simulink model "drone"  (R2026b)
settings: Solver=ode4  StopTime=inf  FixedStep=0.01
values from neighbouring files (symbols this model uses):
  A_d = sys_d.A    [controller_observer_design.m]    (also in setup.m)
  B_d = sys_d.B    [controller_observer_design.m]    (also in setup.m)
  C_d = sys_d.C    [controller_observer_design.m]    (also in setup.m)
  K_discrete = dlqr(A_d,B_d,Q*Ts,R*Ts)    [controller_observer_design.m]    (also in setup.m)
  omega2u = [k, k, k, k; L*k, 0, -L*k, 0; 0, L*k, 0, -L*k; b, -b, b, -b]    [controller_observer_design.m]    (also in notes.m; setup.m)
  parameters =     [parameters.mat]
  Ts = 0.01    [controller_observer_design.m]    (also in setup.m)
  u2omega = (1/(4*b*L*k)) * [b*L, 2*b, 0, L*k; b*L, 0, 2*b, -L*k; b*L, -2*b, 0, L*k; b*L, 0, -2*b, -L*k]    [controller_observer_design.m]    (also in notes.m; setup.m)
undefined symbols (not defined in the file or in its folder): L_discrete
libraries: simulink x2
settings Model: Creator=elton  LastModifiedBy=eltnw

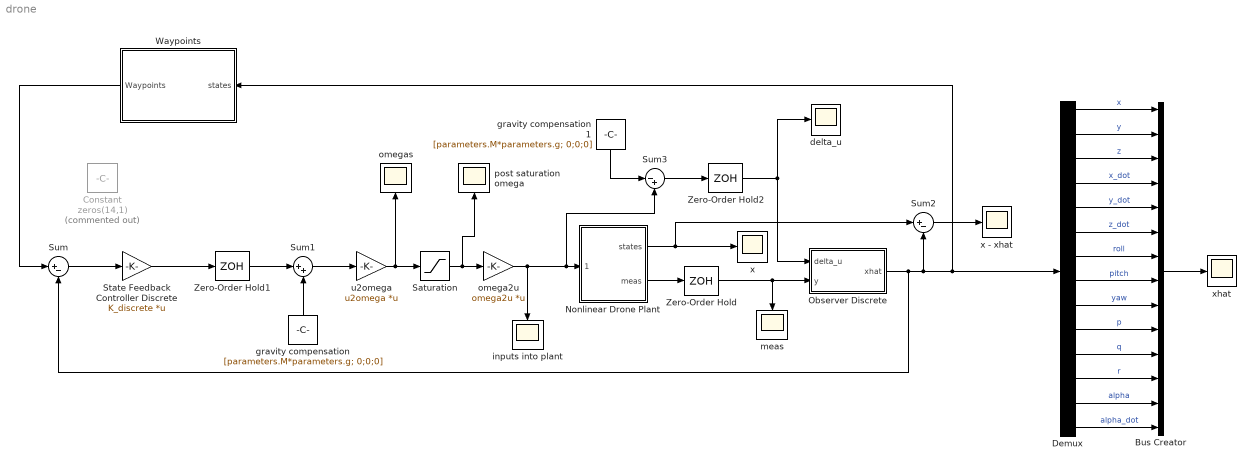
== system drone ==
  Bus Creator : BusCreator  Inputs=14
  Constant : Constant  Commented=on  Value=zeros(14,1)
  Demux : Demux  Outputs=14
  Nonlinear Drone Plant : Subsystem
  Observer Discrete : Subsystem
  Saturation : Saturate  UpperLimit=250000  LowerLimit=-250000
  State Feedback Controller Discrete : Gain  Gain=K_discrete  Multiplication=Matrix(K*u)
  Sum : Sum  Inputs=|+-
  Sum1 : Sum  Inputs=|++
  Sum2 : Sum  Inputs=|+-
  Sum3 : Sum  Inputs=|-+
  Waypoints : Subsystem
  Zero-Order Hold : ZeroOrderHold  SampleTime=Ts
  Zero-Order Hold1 : ZeroOrderHold  SampleTime=Ts
  Zero-Order Hold2 : ZeroOrderHold  SampleTime=Ts
  delta_u : Scope
      settings: ActiveDisplayYMinimum=-0.1401923631580794  ActiveDisplayYMaximum=0.1652403175832419
  gravity compensation : Constant  Value=[parameters.M*parameters.g; 0;0;0]
  gravity compensation1 : Constant  Value=[parameters.M*parameters.g; 0;0;0]
  inputs into plant : Scope
      settings: ActiveDisplayYMinimum=-2.3883084159431922  ActiveDisplayYMaximum=20.39828479264926  DataLoggingVariableName=ScopeData7
  meas : Scope
      settings: ActiveDisplayYMinimum=-955.77756320006051  ActiveDisplayYMaximum=3490.5526217286788
  omega2u : Gain  Gain=omega2u  Multiplication=Matrix(K*u)
  omegas : Scope
      settings: ActiveDisplayYMinimum=-4.7458150182251656E+8  ActiveDisplayYMaximum=6.7744655103517926E+8  DataLoggingVariableName=ScopeData8
  post saturation omega : Scope
      settings: ActiveDisplayYMinimum=-3047.5832245298225  ActiveDisplayYMaximum=278116.39813605888  DataLoggingVariableName=ScopeData9
  u2omega : Gain  Gain=u2omega  Multiplication=Matrix(K*u)
  x : Scope
      settings: ActiveDisplayYMinimum=-2.3057854953189612  ActiveDisplayYMaximum=11.36705971645924  DataLoggingVariableName=ScopeData6
  x - xhat : Scope
      settings: ActiveDisplayYMinimum=-0.016053555537243414  ActiveDisplayYMaximum=0.016145822671605803  DataLoggingVariableName=ScopeData2
  xhat : Scope
      settings: ActiveDisplayYMinimum=-1.314265661412086  ActiveDisplayYMaximum=11.256891286390609  DataLoggingVariableName=ScopeData3
  wires:
  Sum/1 -> State Feedback Controller Discrete/1
  omega2u/1 -> Sum3/2, Nonlinear Drone Plant/1(inputs), inputs into plant/1
  Nonlinear Drone Plant/1(states) -> x/1, Sum2/1
  Zero-Order Hold1/1 -> Sum1/1
  Nonlinear Drone Plant/2(meas) -> Zero-Order Hold/1
  u2omega/1 -> Saturation/1, omegas/1
  Saturation/1 -> post saturation omega/1, omega2u/1
  Zero-Order Hold/1 -> meas/1, Observer Discrete/2(y)
  Zero-Order Hold2/1 -> delta_u/1, Observer Discrete/1(delta_u)
  Observer Discrete/1(xhat) -> Waypoints/1(states), Demux/1, Sum2/2, Sum/2
  Sum2/1 -> x - xhat/1
  gravity compensation/1 -> Sum1/2
  State Feedback Controller Discrete/1 -> Zero-Order Hold1/1
  gravity compensation1/1 -> Sum3/1
  Sum1/1 -> u2omega/1
  Sum3/1 -> Zero-Order Hold2/1
  Waypoints/1(Waypoints) -> Sum/1
  Demux/1 -> Bus Creator/1  "x"
  Demux/2 -> Bus Creator/2  "y"
  Demux/3 -> Bus Creator/3  "z"
  Demux/4 -> Bus Creator/4  "x_dot"
  Demux/5 -> Bus Creator/5  "y_dot"
  Demux/6 -> Bus Creator/6  "z_dot"
  Demux/7 -> Bus Creator/7  "roll"
  Demux/8 -> Bus Creator/8  "pitch"
  Demux/9 -> Bus Creator/9  "yaw"
  Demux/10 -> Bus Creator/10  "p"
  Demux/11 -> Bus Creator/11  "q"
  Demux/12 -> Bus Creator/12  "r"
  Demux/13 -> Bus Creator/13  "alpha"
  Demux/14 -> Bus Creator/14  "alpha_dot"
  Bus Creator/1 -> xhat/1

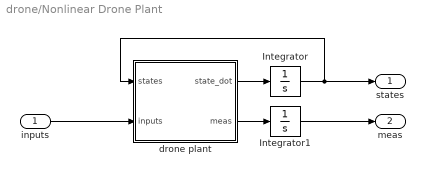
== system drone/Nonlinear Drone Plant ==
  inputs : Inport
  Integrator : Integrator  InitialCondition=[zeros(12,1); 0; 0]
  Integrator1 : Integrator  InitialCondition=zeros(6,1)
  drone plant : MATLAB Function  TreatAsAtomicUnit=on
  states : Outport
  meas : Outport  Port=2
  wires:
  drone plant/1(state_dot) -> Integrator/1
  Integrator/1 -> states/1, drone plant/1(states)
  inputs/1 -> drone plant/2(inputs)
  Integrator1/1 -> meas/1
  drone plant/2(meas) -> Integrator1/1

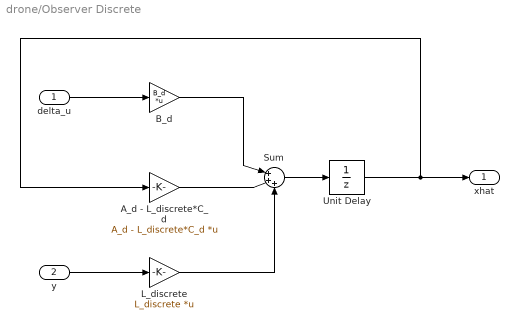
== system drone/Observer Discrete ==
  delta_u : Inport
  y : Inport  Port=2
  A_d - L_discrete*C_d : Gain  Gain=A_d - L_discrete*C_d  Multiplication=Matrix(K*u)
  B_d : Gain  Gain=B_d  Multiplication=Matrix(K*u)
  L_discrete : Gain  Gain=L_discrete  Multiplication=Matrix(K*u)
  Sum : Sum  Inputs=|+++
  Unit Delay : UnitDelay  InitialCondition=zeros(14,1)  SampleTime=-1
  xhat : Outport
  wires:
  y/1 -> L_discrete/1
  B_d/1 -> Sum/1
  L_discrete/1 -> Sum/3
  A_d - L_discrete*C_d/1 -> Sum/2
  Sum/1 -> Unit Delay/1
  Unit Delay/1 -> A_d - L_discrete*C_d/1, xhat/1
  delta_u/1 -> B_d/1

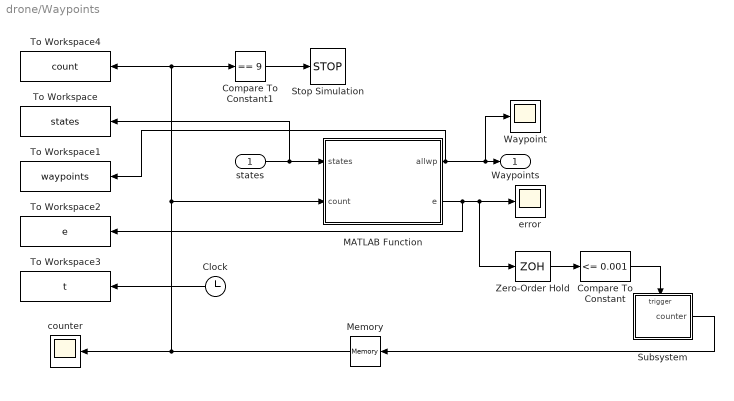
== system drone/Waypoints ==
  states : Inport
  Clock : Clock
  Compare To Constant : simulink/Logic and Bit Operations/Compare To Constant  relop=<=  const=0.001  OutDataTypeStr=boolean
  Compare To Constant1 : simulink/Logic and Bit Operations/Compare To Constant  relop===  const=9  OutDataTypeStr=boolean
  MATLAB Function : MATLAB Function  TreatAsAtomicUnit=on
  Memory : Memory  InheritSampleTime=on
  Stop Simulation : Stop
  Subsystem : Subsystem
  To Workspace : ToWorkspace  VariableName=states  SampleTime=-1
  To Workspace1 : ToWorkspace  VariableName=waypoints  SampleTime=-1
  To Workspace2 : ToWorkspace  VariableName=e  SampleTime=-1
  To Workspace3 : ToWorkspace  VariableName=t  SampleTime=-1
  To Workspace4 : ToWorkspace  VariableName=count  SampleTime=-1
  Waypoint : Scope
      settings: DataLoggingVariableName=ScopeData4
  Zero-Order Hold : ZeroOrderHold  SampleTime=0.01
  counter : Scope
      settings: DataLoggingVariableName=ScopeData5
  error : Scope
      settings: ActiveDisplayYMinimum=-0.89185486903848621  ActiveDisplayYMaximum=8.0341746816232842  DataLoggingVariableName=ScopeData10
  Waypoints : Outport
  wires:
  Compare To Constant/1 -> Subsystem/Trigger
  Memory/1 -> Compare To Constant1/1, To Workspace4/1, MATLAB Function/2(count), counter/1
  MATLAB Function/2(e) -> To Workspace2/1, Zero-Order Hold/1, error/1
  states/1 -> To Workspace/1, MATLAB Function/1(states)
  Subsystem/1(counter) -> Memory/1
  Zero-Order Hold/1 -> Compare To Constant/1
  Clock/1 -> To Workspace3/1
  MATLAB Function/1(allwp) -> To Workspace1/1, Waypoint/1, Waypoints/1
  Compare To Constant1/1 -> Stop Simulation/1

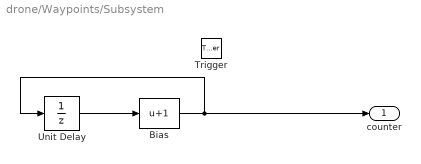
== system drone/Waypoints/Subsystem ==
  Trigger : TriggerPort  VariantControl=(inherit)  InitialTriggerSignalState=positive  PortDimensions=1
  Bias : Bias  Bias=1  SaturateOnIntegerOverflow=off
  Unit Delay : UnitDelay  SampleTime=-1
  counter : Outport
  wires:
  Unit Delay/1 -> Bias/1
  Bias/1 -> Unit Delay/1, counter/1

== matlab function drone/Waypoints/MATLAB Function ==
  data: states input; allwp output; count input; e output
function [allwp, e] = waypoints(states, count)
wps0 = [5 8 8 7 9 6 3 3;
    1 3 2 9 6 5 8 2;
    1 5 9 10 5 4 3 3];

%wps0 = [4 10 0 1 7 2 8 10;
        %2 9 8 5 2 1 8 9;
        %8 4 9 7 5 3 1 1];
persistent wps
if isempty(wps)
    wps = shortestTour(wps0, zeros(3,1), zeros(3,1));
end
%wps = wps0;
xi = states(1:3);
wp = zeros(3,1);
if count < size(wps, 2)
    wp = wps(:, uint8(count+1));
end
e = norm(xi - wp);
d_max = 0.7;
err  = wp - xi;
dist = norm(err);
if dist > d_max
    ref = xi + d_max * err / dist;
else
    ref = wp;
end
allwp = zeros(14,1);
allwp(1:3) = ref;
end

function out = shortestTour(P, startPt, endPt)
N  = size(P, 2);
nm = 2^N;

D = zeros(N, N);
for i = 1:N
    for j = 1:N
        D(i,j) = norm(P(:,i) - P(:,j));
    end
end

% Length of the order as entered
givenLen = norm(P(:,1) - startPt) + norm(P(:,N) - endPt);
for i = 1:N-1
    givenLen = givenLen + D(i,i+1);
end

% Held-Karp: exact shortest path start -> all points -> end
cost   = inf(nm, N);
parent = zeros(nm, N);
for j = 1:N
    cost(2^(j-1) + 1, j) = norm(P(:,j) - startPt);
end
for mask = 1:nm-1
    for j = 1:N
        if bitand(mask, 2^(j-1)) == 0 || isinf(cost(mask+1, j))
            continue;
        end
        for k = 1:N
            if bitand(mask, 2^(k-1)) ~= 0
                continue;
            end
            nmask = mask + 2^(k-1);
            c = cost(mask+1, j) + D(j,k);
            if c < cost(nmask+1, k)
                cost(nmask+1, k)   = c;
                parent(nmask+1, k) = j;
            end
        end
    end
end

allMask = nm - 1;
best = inf;
last = 1;
for j = 1:N
    c = cost(allMask+1, j) + norm(P(:,j) - endPt);
    if c < best
        best = c;
        last = j;
    end
end

% Already shortest (including ties)? Keep the entered order.
if givenLen <= best + 1e-9
    out = P;
    return;
end

order = zeros(1, N);
mask  = allMask;
j     = last;
for idx = N:-1:1
    order(idx) = j;
    pj   = parent(mask+1, j);
    mask = mask - 2^(j-1);
    j    = pj;
end
out = P(:, order);
end

== matlab function drone/Nonlinear Drone Plant/drone plant ==
  data: states input size=14; inputs input size=4; state_dot output size=14; parameters parameter; meas output
%% non-linear state space
function [state_dot, meas]  = nonlin_state_space(states, inputs, parameters)
m     = parameters.m;
m_p    = parameters.m_p;
M     = m + m_p;
g     = parameters.g;
l     = parameters.l;
k_D    = parameters.k_D;
I_xx  = parameters.I_xx;
I_yy  = parameters.I_yy;
I_zz  = parameters.I_zz;

xi = states(1:3);
xi_dot = states(4:6);
eta = states(7:9);
nu = states(10:12);
alpha = states(13);
alpha_dot = states(14);

u_T = inputs(1);
tau = inputs(2:4);

x_dot = xi_dot(1);
y_dot = xi_dot(2);
z_dot = xi_dot(3);

% kinematics
phi = eta(1);
theta = eta(2);
psi = eta(3);
W_inv = [1,  sin(phi)*tan(theta), cos(phi)*tan(theta);
    0,  cos(phi),            -sin(phi);
    0,  sin(phi)/cos(theta), cos(phi)/cos(theta)];

eta_dot = W_inv*nu;

%rotational dynamics
p_dot = (tau(1)/I_xx) + ((I_yy-I_zz)/I_xx)*nu(2)*nu(3);
q_dot = (tau(2)/I_yy) + ((I_zz-I_xx)/I_yy)*nu(1)*nu(3);
r_dot = (tau(3)/I_zz) + ((I_xx-I_yy)/I_zz)*nu(1)*nu(2);
nu_dot = [p_dot; q_dot; r_dot];

%translational dynamics
c_alpha = cos(alpha);
s_alpha = sin(alpha);
c_phi = cos(phi); s_phi = sin(phi);
c_theta = cos(theta); s_theta = sin(theta);
c_psi = cos(psi); s_psi = sin(psi);

Fx = (c_psi*s_theta*c_phi + s_psi*s_phi) * u_T;
Fy = (s_psi*s_theta*c_phi - c_psi*s_phi) * u_T;
Fz = c_theta*c_phi * u_T;

x_dotdot = (1/(m*M)) * ( (m + m_p*c_alpha^2)*(Fx - k_D*x_dot) - m_p*s_alpha*c_alpha*(Fz - k_D*z_dot) + m*m_p*l*alpha_dot^2*s_alpha );
y_dotdot = (Fy - k_D*y_dot) / m;
z_dotdot = (1/(m*M)) * ( (m + m_p*s_alpha^2)*(Fz - k_D*z_dot) - m_p*s_alpha*c_alpha*(Fx - k_D*x_dot) + m*m_p*l*alpha_dot^2*c_alpha ) - g;
xi_dotdot = [x_dotdot; y_dotdot; z_dotdot];

% pendulum dynamics
%alpha_dotdot = (1 / (M * l)) * ( -Fx * c_alpha + Fz * s_alpha + k_D * x_dot * c_alpha - k_D * z_dot * s_alpha );
alpha_dotdot = (1/l)*(-x_dotdot*c_alpha - z_dotdot*s_alpha+g*s_alpha);

% assemble state_dot and meas
state_dot = [xi_dot; xi_dotdot; eta_dot; nu_dot; alpha_dot; alpha_dotdot];
meas = [xi_dot; eta_dot];
end
